simulink model "SZ10_JB"  (R2026a)
settings: Solver=VariableStepAuto  StopTime=2  MaxStep=0.002
settings Model: Creator=Szalay  LastModifiedBy=Szalay

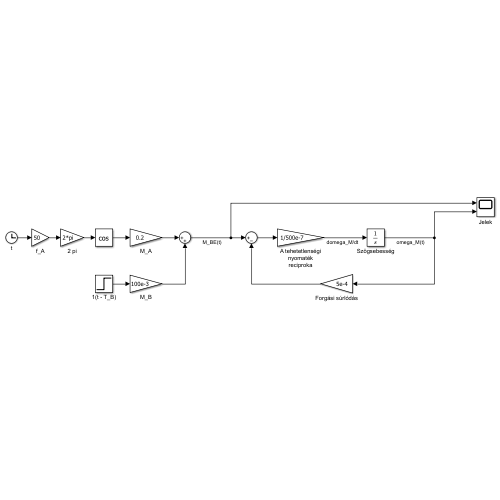
[thumbnail: Simulink's stored preview of the top-level diagram]
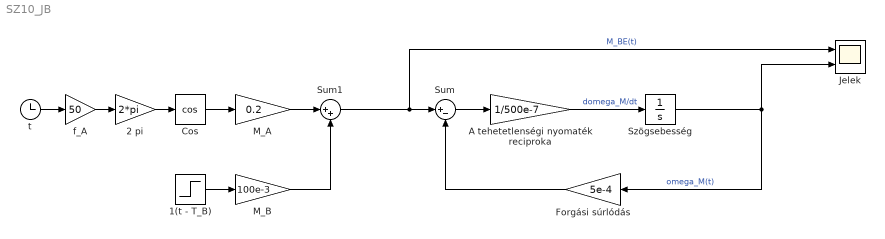
== system SZ10_JB ==
  1(t - T_B) : Step  Time=1250e-3  SampleTime=0
  2 pi : Gain  Gain=2*pi
  A tehetetlenségi nyomaték reciproka : Gain  Gain=1/500e-7
  Cos : Trigonometry  Operator=cos
  Forgási súrlódás : Gain  Gain=5e-4
  Jelek : Scope  NumInputPorts=2
      settings: ActiveDisplayYMinimum=-40.260886899598482  ActiveDisplayYMaximum=240.13151259249329
  M_A : Gain  Gain=0.2
  M_B : Gain  Gain=100e-3
  Sum : Sum  Inputs=|+-
  Sum1 : Sum  Inputs=|++
  Szögsebesség : Integrator  InitialCondition=100
  f_A : Gain  Gain=50
  t : Clock
  wires:
  Szögsebesség/1 -> Jelek/2, Forgási súrlódás/1  "omega_M(t)"
  A tehetetlenségi nyomaték reciproka/1 -> Szögsebesség/1  "domega_M/dt"
  Sum/1 -> A tehetetlenségi nyomaték reciproka/1
  Forgási súrlódás/1 -> Sum/2
  Sum1/1 -> Jelek/1, Sum/1  "M_BE(t)"
  Cos/1 -> M_A/1
  M_A/1 -> Sum1/1
  2 pi/1 -> Cos/1
  f_A/1 -> 2 pi/1
  t/1 -> f_A/1
  1(t - T_B)/1 -> M_B/1
  M_B/1 -> Sum1/2
